simulink subsystem "ReactionWheel"  (R2024b)
settings: Solver=VariableStepAuto  StartTime=0.0  StopTime=10.0  RelTol=1e-3
model mask{k=0, maxSpeed=0, capacity=0, imbalance=0, R=0, seed=0, torqueVariance=0}
  mask prompts: k "Scale factor"; maxSpeed "Max Speed"; imbalance "Wheel imbalance"; R "Rotation Matrix"; torqueVariance "Torque Variance"
libraries: matrix_library x1
settings Model: Creator=marco  LastModifiedBy=ferru

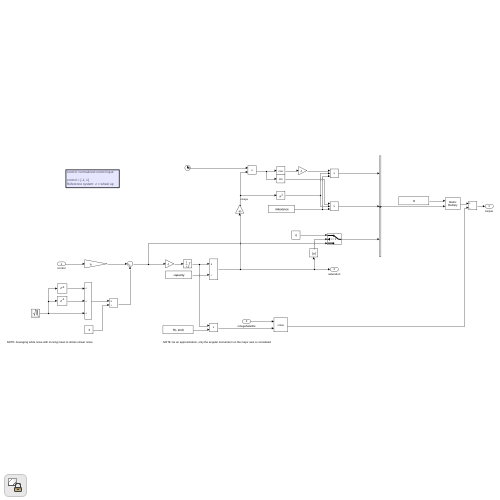
[thumbnail: Simulink's stored preview of the top-level diagram]
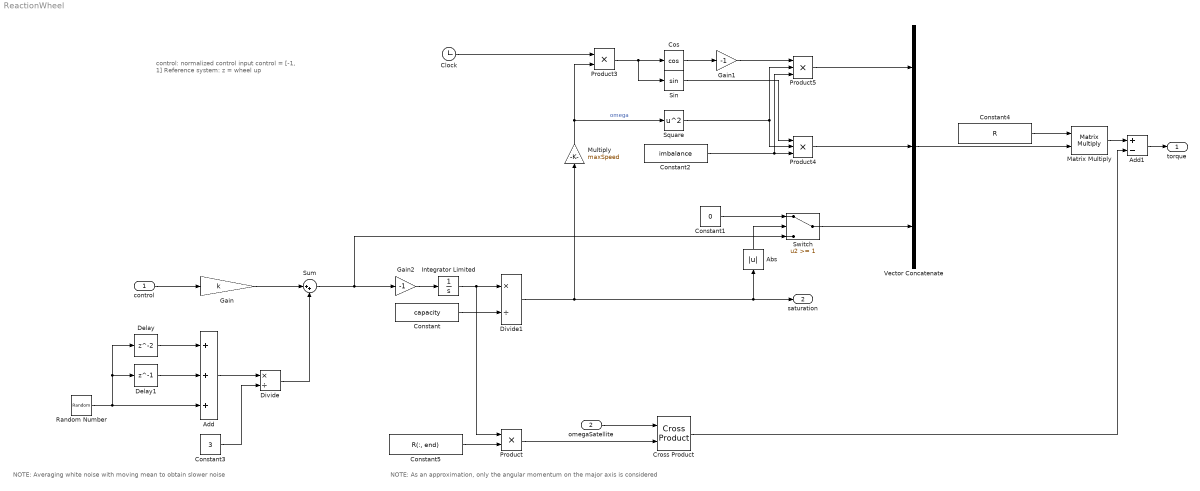
== system ReactionWheel ==
  note: NOTE: As an approximation, only the angular momentum on the major axis is considered
  note: NOTE: Averaging white noise with moving mean to obtain slower noise
  note: control: normalized control input
      |
      | control = [-1, 1]
      | Reference system: z = wheel up
  control : Inport  OutMin=-1  OutMax=1
  omegaSatellite : Inport  Port=2
  Abs : Abs  SaturateOnIntegerOverflow=off
  Add : Sum  Inputs=3
  Add1 : Sum  Inputs=+-
  Clock : Clock
  Constant : Constant  Value=capacity
  Constant1 : Constant  Value=0
  Constant2 : Constant  Value=imbalance
  Constant3 : Constant  Value=3
  Constant4 : Constant  Value=R  VectorParams1D=off
  Constant5 : Constant  Value=R(:, end)  VectorParams1D=off
  Cos : Trigonometry  Operator=cos
  Cross Product : matrix_library/Cross Product
  Delay : Delay
  Delay1 : Delay  DelayLength=1
  Divide : Product  Inputs=*/
  Divide1 : Product  Inputs=*/
  Gain : Gain  Gain=k
  Gain1 : Gain  Gain=-1
  Gain2 : Gain  Gain=-1
  Integrator Limited : Integrator  LimitOutput=on  UpperSaturationLimit=capacity  LowerSaturationLimit=-capacity
  Matrix Multiply : Product  Multiplication=Matrix(*)
  Multiply : Gain  Gain=maxSpeed
  Product : Product
  Product3 : Product
  Product4 : Product  Inputs=3
  Product5 : Product  Inputs=3
  Random Number : RandomNumber  Variance=torqueVariance  Seed=seed + 1
  Sin : Trigonometry
  Square : Math  Operator=square
  Sum : Sum  Inputs=|++
  Switch : Switch  Threshold=1  SaturateOnIntegerOverflow=off  InputSameDT=off
  Vector Concatenate : Concatenate  NumInputs=3  Mode=Multidimensional array
  torque : Outport
  saturation : Outport  Port=2
  wires:
  control/1 -> Gain/1
  Integrator Limited/1 -> Divide1/1, Product/1
  Clock/1 -> Product3/1
  Product3/1 -> Sin/1, Cos/1
  Cos/1 -> Gain1/1
  Sin/1 -> Product4/1
  Square/1 -> Product5/2, Product4/2
  Constant2/1 -> Product4/3, Product5/3
  Gain1/1 -> Product5/1
  Product5/1 -> Vector Concatenate/1
  Product4/1 -> Vector Concatenate/2
  Sum/1 -> Switch/3, Gain2/1
  Divide1/1 -> Multiply/1, saturation/1, Abs/1
  Constant/1 -> Divide1/2
  Multiply/1 -> Square/1, Product3/2  "omega"
  Constant1/1 -> Switch/1
  Switch/1 -> Vector Concatenate/3
  Vector Concatenate/1 -> Matrix Multiply/2
  Constant4/1 -> Matrix Multiply/1
  Matrix Multiply/1 -> Add1/1
  Random Number/1 -> Delay/1, Delay1/1, Add/3
  Delay1/1 -> Add/2
  Delay/1 -> Add/1
  Add/1 -> Divide/1
  Constant3/1 -> Divide/2
  Divide/1 -> Sum/2
  Gain/1 -> Sum/1
  omegaSatellite/1 -> Cross Product/1
  Constant5/1 -> Product/2
  Product/1 -> Cross Product/2
  Cross Product/1 -> Add1/2
  Add1/1 -> torque/1
  Abs/1 -> Switch/2
  Gain2/1 -> Integrator Limited/1
